simulink subsystem "BadMembrane"  (R2025b)
settings: Solver=VariableStepAuto  StartTime=0.0  StopTime=10.0  RelTol=1e-3
libraries: customization_lib x2
settings Model: Creator=ndegoede  LastModifiedBy=degoeden

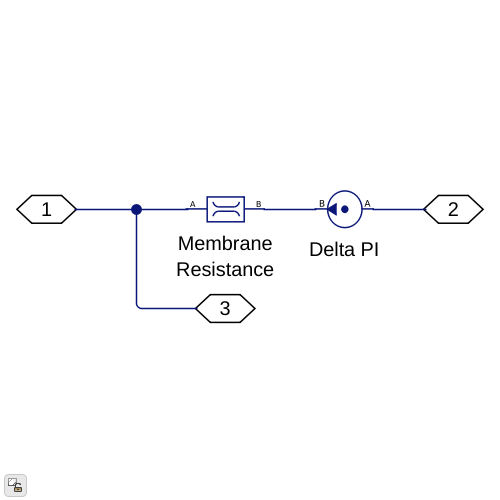
[thumbnail: Simulink's stored preview of the top-level diagram]
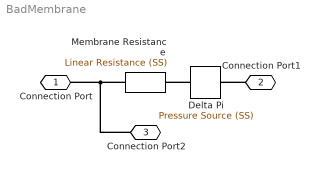
== system BadMembrane ==
  Delta Pi : customization_lib/solution/sources/Pressure Source (SS)  source_type=foundation.enum.constant_controlled.constant  pressure_differential=2.7773 MPa  power_spec=foundation.enum.power_spec.isentropic  area=0.01 m^2  custom_ports=true  length_A=1 m  length_B=1 m
      settings: SourceProductName=Customization  InternalSimscapePortConfiguration="{\"Bottom\":[],\"Left\":[{\"id\":\"A\",\"label\":\"A\",\"type\":\"customization.solution.solution\"}],\"Right\":[{\"id\":\"B\",\"label\":\"B\",\"type\":\"customization.solution.solution\"}],\"Top\":[]}"
  Membrane Resistance : customization_lib/solution/elements/Linear Resistance (SS)  R=6.0986e+07 Pa*s/m^3  area=0.1 m^2  custom_ports=true  length_A=1 m  length_B=1 m
      settings: SourceProductName=Customization  InternalSimscapePortConfiguration="{\"Bottom\":[],\"Left\":[{\"id\":\"A\",\"label\":\"A\",\"type\":\"customization.solution.solution\"}],\"Right\":[{\"id\":\"B\",\"label\":\"B\",\"type\":\"customization.solution.solution\"}],\"Top\":[]}"
  Connection Port : PMIOPort  Side=Left
  Connection Port1 : PMIOPort  Port=2  Side=Left
  Connection Port2 : PMIOPort  Port=3  Side=Left
  connections:
  Membrane Resistance/LConn1 -- Connection Port2/RConn1 -- Connection Port/RConn1
  Connection Port1/RConn1 -- Delta Pi/LConn1
  Delta Pi/RConn1 -- Membrane Resistance/RConn1
